simulink model "aBaja2026"  (R2026a)
settings: Solver=FixedStepAuto  StartTime=0  StopTime=1000  FixedStep=timeStep
PostLoadFcn:
  | helperSLTrajectoryFollowerWithRRScenarioSetup
InitFcn:
  | helperSLTrajectoryFollowerWithRRScenarioSetup
  | worldActor=rrSim.getScenario();
  | world = worldActor.actor_spec.world_spec;
  | % Inputs you already have (example):
  | EgoActorID  = 1;
  | egoSetSpeed = 0;
  | 
  | % Get world + actors
  | 
  | 
  | % --- Find the ego actor (vectorized, minimal overhead) ---
  | actorIDs = arrayfun(@(a) str2double(a.actor_runtime.id), world.actors);
  | idx = (actorIDs == EgoActorID);
  | 
  | if nnz(idx) ~= 1
  |     error("Actor with ActorID:%d does not exist (or is not unique).", EgoActorID);
  | end
  | 
  | ego = world.actors(idx);
  | 
  | % --- Build 4x4 pose matrix quickly ---
  | temp_m = ego.actor_runtime.pose.matrix;
  | pose = [temp_m.col0.x temp_m.col1.x temp_m.col2.x temp_m.col3.x; ...
  |         temp_m.col0.y temp_m.col1.y temp_m.col2.y temp_m.col3.y; ...
  |         temp_m.col0.z temp_m.col1.z temp_m.col2.z temp_m.col3.z; ...
  |         temp_m.col0.w temp_m.col1.w temp_m.col2.w temp_m.col3.w];
  | 
  | rotm = pose(1:3,1:3);
  | pos  = pose(1:3,4)';   % [x y z] meters
  | 
  | % --- Euler angles from rotation matrix (ZYX: yaw, pitch, roll) ---
  | % If you have Robotics System Toolbox, rotm2eul exists; otherwise keep internal.
  | if exist("rotm2eul","file")
  |     eulZYX = rotm2eul(rotm,"ZYX");                 % radians: [yaw pitch roll]
  | else
  |     eulZYX = robotics.internal.rotm2eul(rotm,"ZYX");% radians: [yaw pitch roll]
  | end
  | 
  | % RoadRunner yaw -> conventional yaw:
  | yawDeg   = rad2deg(eulZYX(1)) + 90;
  | yawDeg   = mod(yawDeg + 180, 360) - 180;           % wrap to (-180,180]
  | pitchDeg = rad2deg(eulZYX(2));
  | rollDeg  = rad2deg(eulZYX(3));
  | 
  | % --- (Optional) reproduce your actorPose struct (kept consistent) ---
  | vGlobal = [egoSetSpeed*cosd(yawDeg), egoSetSpeed*sind(yawDeg), 0];
  | vBody   = (rotm' * vGlobal')';                      % body-fixed velocity
  | 
  | actorPose = struct( ...
  |     'ActorID', double(EgoActorID), ...
  |     'Position', pos, ...
  |     'Velocity', vGlobal, ...
  |     'vehicleFrameVelocity', [vBody(2), -vBody(1), vBody(3)], ...
  |     'Roll',  rollDeg, ...
  |     'Pitch', pitchDeg, ...
  |     'Yaw',   yawDeg, ...
  |     'AngularVelocity', [0 0 0]);
  | 
  | % --- Inline replacement for poseToSim3DInputs ---
  | % IMPORTANT: your original poseToSim3DInputs uses radians (pi terms),
  | ... (+13 lines)
undefined symbols (not defined in the file): Defined, Ego, Lane, LKA, m, matlabshared, n, Pose, Sim3dSensor, timeStep, User, Velocity
libraries: roadrunnerscenario x9, drivingvehiclecontroller x3, simulink_extras x3, sim3dautolib x2, drivingscenarioandsensors x1, sim3dcameralib x1, sim3dlib x1, simulink x1
(part 2 of 2)

== system aBaja2026/LKA (Lane Keeping Assist)/Lane Source/Camera Lane Detector/Vision Lane Detector ==
  Image : Inport
  Lane Detector : MATLABSystem  System=LkaVisionLaneDetector  Vision=LKA.Vision  Ts=LKA.Ts
      mask Type: LkaVisionLaneDetector
  Processing Latency : Delay  DelayLength=LKA.Vision.LatencySteps  InitialCondition=0  SampleTime=LKA.Ts
  LaneSensor : Outport  OutDataTypeStr=Bus: LaneSensorBus
  Preview : Outport  Port=2
  VisionInfo : Outport  Port=3
  wires:
  Image/1 -> Lane Detector/1
  Lane Detector/1 -> Processing Latency/1
  Processing Latency/1 -> LaneSensor/1
  Lane Detector/2 -> Preview/1
  Lane Detector/3 -> VisionInfo/1

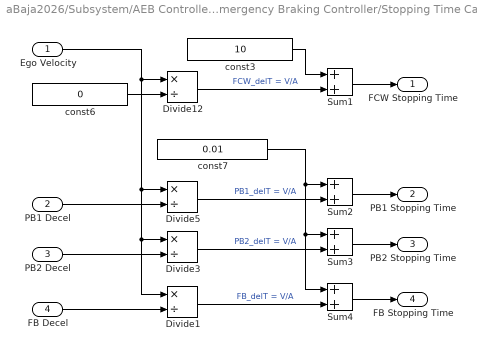
== system aBaja2026/Subsystem/AEB Controller/Emergency Braking Controller/Stopping Time Calculation ==
  Ego Velocity : Inport  SampleTime=timeStep
  PB1 Decel : Inport  Port=2
  PB2 Decel : Inport  Port=3
  FB Decel : Inport  Port=4
  Divide{1,3,5,12} (4 alike) : Product  Inputs=*/
  Sum{1..4} (4 alike) : Sum
  const3 : Constant  Value=10  SampleTime=-1
  const6 : Constant  Value=0  SampleTime=-1
  const7 : Constant  Value=0.01  SampleTime=-1
  FCW Stopping Time : Outport  VectorParamsAs1DForOutWhenUnconnected=off
  PB1 Stopping Time : Outport  Port=2  VectorParamsAs1DForOutWhenUnconnected=off
  PB2 Stopping Time : Outport  Port=3  VectorParamsAs1DForOutWhenUnconnected=off
  FB Stopping Time : Outport  Port=4  VectorParamsAs1DForOutWhenUnconnected=off
  wires:
  Sum1/1 -> FCW Stopping Time/1
  Sum2/1 -> PB1 Stopping Time/1
  Sum3/1 -> PB2 Stopping Time/1
  Sum4/1 -> FB Stopping Time/1
  const7/1 -> Sum2/1, Sum4/1, Sum3/1
  Ego Velocity/1 -> Divide1/1, Divide3/1, Divide5/1, Divide12/1
  Divide5/1 -> Sum2/2  "PB1_delT = V/A"
  Divide3/1 -> Sum3/2  "PB2_delT = V/A"
  Divide1/1 -> Sum4/2  "FB_delT = V/A"
  const6/1 -> Divide12/2
  PB1 Decel/1 -> Divide5/2
  PB2 Decel/1 -> Divide3/2
  FB Decel/1 -> Divide1/2
  const3/1 -> Sum1/1
  Divide12/1 -> Sum1/2  "FCW_delT = V/A"

== system aBaja2026/Subsystem/AEB Controller/Emergency Braking Controller/TTC Calculation ==
  Mio Distance : Inport
  Mio Velocity : Inport  Port=2
  Abs : Abs  SaturateOnIntegerOverflow=off
  Divide11 : Product  Inputs=**
  Divide3 : Product  Inputs=*/
  Saturation : Saturate  UpperLimit=100  LowerLimit=0.01
  Sign : Signum
  Sum : Sum  Inputs=+-
  const1 : Constant  Value=0  SampleTime=-1
  TTC : Outport  VectorParamsAs1DForOutWhenUnconnected=off
  wires:
  Mio Velocity/1 -> Sign/1, Abs/1
  Mio Distance/1 -> Sum/1
  Divide3/1 -> Divide11/1  "TTC"
  const1/1 -> Sum/2
  Sum/1 -> Divide3/1  "headway"
  Abs/1 -> Saturation/1
  Saturation/1 -> Divide3/2
  Sign/1 -> Divide11/2
  Divide11/1 -> TTC/1

== matlab function aBaja2026/Subsystem2/MATLAB Function1 ==
  data: T input; Translation output; Rotation output
function [Translation, Rotation] = poseToSim3DInputs(T)
% T: 4x4 pose matrix
% Outputs:
%   Translation - 5x3 matrix
%   Rotation    - 5x3 matrix

% ------------------------------------------
% 1. Extract vehicle translation
% ------------------------------------------
Xv = T(1,4);
Yv = -1*T(2,4);
Zv = T(3,4);

% ------------------------------------------
% 2. Extract vehicle yaw (ISO 8855, Z-down)
% ------------------------------------------
yaw = atan2(T(2,1), T(1,1));    % heading
roll = 0;                       % assume level (modify if needed)
pitch = 0;

% ------------------------------------------
% 3. Build Translation 5×3
% Row 1 = vehicle
% Rows 2–5 = wheels (zero unless user fills)
% ------------------------------------------
Translation = zeros(5,3);
Translation(1,:) = [Xv, Yv, Zv];

% ------------------------------------------
% 4. Build Rotation 5×3
% Row 1 = vehicle rotation
% Rows 2–5 = wheels
% ------------------------------------------
Rotation = zeros(5,3);
Rotation(1,:) = [roll, pitch, -yaw+pi/2+pi];

== matlab function aBaja2026/Subsystem2/Pack Actor Pose/Velocity XYZ Components ==
  data: yaw input size=1; velocity output size=[1 3]; speed input size=1
function velocity = computeVelocity(yaw, speed)

% Output velocity vector (x,y,z)
velocity = speed * [-sind(yaw) cosd(yaw) 0];

== matlab function aBaja2026/Subsystem2/Lateral Metrics ==
  data: currPose input size=[1 3]; refPose input size=[1 3]; positionError output; headingError output
function [positionError, headingError] = lateralMetrics(currPose, refPose)
%lateralMetrics calculates lateral error and heading error of the vehicle 
% using current and reference pose

currPose(:,3) = deg2rad(currPose(:,3));
refPose(:,3)  = deg2rad(refPose(:,3));

positionError = norm(currPose(1:2) - refPose(1:2));

headingError = rad2deg(currPose(:, 3) - refPose(:,3));

== matlab function aBaja2026/LKA (Lane Keeping Assist)/Skeleton Pose Adapter ==
  data: veh input Bus: BusVehicleInfo; egoPose output; refPose input; refCurv input; mode input; centerPose output; curv output; speed output; yawRate output; enable output; yawRatePose output; LKA parameter
function [egoPose, centerPose, curv, speed, yawRate, enable, yawRatePose] = fcn(veh, refPose, refCurv, mode, LKA)
% Skeleton signals -> LKA conventions (SI units, radians, rear-axle reference).
% speed / yawRate stand for the wheel-speed sensor and the gyro (noise added by the
% Ego Sensors block). egoPose, centerPose, curv feed only the emulated sensor
% (development variant). yawRatePose is differentiated from the ground-truth pose
% and only logged to verify LKA.Cosim.YawRateSign (rule I.2.3: not a controller input).
persistent psiPrev
psi = deg2rad(veh.CurrPose(3) + LKA.Cosim.YawOffsetDeg);
if isempty(psiPrev), psiPrev = psi; end
yawRatePose = lka_wrap_angle(psi - psiPrev) / LKA.Ts;
psiPrev = psi;
yawRate = LKA.Cosim.YawRateSign * deg2rad(veh.CurrYawRate);
egoPose = [veh.CurrPose(1) + LKA.Cosim.PoseToRearAxle*cos(psi), ...
           veh.CurrPose(2) + LKA.Cosim.PoseToRearAxle*sin(psi), psi];
centerPose = [refPose(1), refPose(2), deg2rad(refPose(3) + LKA.Cosim.YawOffsetDeg)];
curv = [refCurv(1), 0];
speed = abs(veh.CurrVelocity);
enable = any(mode == LKA.Cosim.LkaModes);

== matlab function aBaja2026/Subsystem2/Initialize State/Calculate Initial States/Calculate Initial States ==
  data: egoRuntime input; egoInitialState output Bus: BusVehicleInfo
function egoInitialState = getInitialState(egoRuntime)
%getInitialState calculates initial conditions of the vehicle

% Calculate velocity
velocity = norm(egoRuntime.ActorRuntime.Velocity,2);
% Get Transformation matrix
transformationMatrix = egoRuntime.ActorRuntime.Pose;
% Get pose information
x = transformationMatrix(1,4);
y = transformationMatrix(2,4);
yaw = atan2d(-transformationMatrix(1,2), ...
            transformationMatrix(1,1));
% Pack the initial states
egoInitialState = struct('CurrPose', [y, -x, yaw], ...
    'CurrVelocity', velocity, ...
    'CurrYawRate', 0, ...
    'CurrSteer',0, ...
    'Direction',1);

== matlab function aBaja2026/Subsystem/AEB Controller/Ego Speed ==
  data: speed output; velocity input
function speed = egoSpeed(velocity)

speed = norm([velocity(1), velocity(2), velocity(3)]);

== stateflow chart aBaja2026/Subsystem/AEB Controller/Emergency Braking Controller/AEB Logic ==
  note: FCW/AEB Logic
  state Default
    entry: AEBstatus = 0;
    FCWactivate = 0;
    decel = 0;
  state FCW
    entry: AEBstatus = 0;
    FCWactivate = 1;
    decel = 0;
  state Partial_Braking1
    entry: AEBstatus = 1;
    FCWactivate = 1;
    decel = PB1decel;
  state Full_Braking
    entry: AEBstatus = 3;
    FCWactivate = 1;
    decel = FBdecel;
  state Partial_Braking2
    entry: AEBstatus = 2;
    FCWactivate = 1;
    decel = PB2decel;
  (default) -> Default
  (junction 78) -> Default
  Full_Braking -> (junction 78) [order 1] : [stop==1]
  (junction 80) -> Default
  (junction 90) -> (junction 80) : [stop==1]
  (junction 86) -> Default
  (junction 88) -> (junction 86)
  Default -> FCW : [(abs(TTC)<FCWtime) && TTC<0&&stop~=1]
  FCW -> (junction 76) [order 1]
  (junction 76) -> Full_Braking : [ abs(relativeYawAngle) >= deg2rad(89) && TTC<0 && ...
      | stop~=1]
  FCW -> Partial_Braking1 [order 2] : [(abs(TTC) < PB1time) && TTC<0&&stop~=1]
  Partial_Braking1 -> (junction 88) [order 2] : [stop==1]
  Partial_Braking1 -> Partial_Braking2 [order 1] : [(abs(TTC) < PB2time) && TTC<0&&stop~=1]
  Partial_Braking2 -> Partial_Braking1 [order 2] : [abs(TTC)>=1.2*PB2time]
  Partial_Braking2 -> (junction 90) [order 1]
  Full_Braking -> Partial_Braking2 [order 2] : [abs(TTC)>=3*FBtime]
  Partial_Braking2 -> Full_Braking [order 3] : [(abs(TTC) < FBtime) && TTC<0&&stop~=1]
  data: FCWactivate output uint8; TTC input; FCWtime input; PB1time input; PB2time input; FBtime input; PB1decel input; PB2decel input; FBdecel input; AEBstatus output uint8; decel output; stop input; relativeYawAngle input

== matlab function aBaja2026/Subsystem/AEB Controller/Find MIO ==
  data: confirmedTracks input size=[1 1]; x output size=[1 1]; vx output size=[1 1]; positionSelector input; laneWidth input; relativeYawAngle output double size=[1 1]; egoSpeed input double size=[1 1]
function [x,vx, relativeYawAngle] = findMIO(confirmedTracks, positionSelector, laneWidth, egoSpeed)
% This function finds the lead car: a car in front of the ego car that
% satisfies all the criteria below:
% * Within the ego car's lane.
% * In front of the ego car.
% * Closest to the ego car.

% Important notes:
% 1. If you change state definition, change the following:
%       State = [x;vx;y;vy;z;vz] (3D constant velocity)
numStates = 6;
relativeYawAngle =0 ;
% 2. The ego car is assumed to be traveling in the middle of its lane.
halfLaneWidth = laneWidth/2;

% Initialize outputs and parameters
maxX = cast(1000, 'like', confirmedTracks.Tracks(1).State);  % Far enough forward so that no track is expected to exceed this distance
trackID = 0;
crossingTargetLateralDist = 18;
targetCollisionThresholdTime = 2; % Collision threshold time beyond which the target should be treated as MIO 
stationaryVelocityThreshold = eps('single'); % Threshold to determine if a target is effectively stationary relative to the world

for i = 1:confirmedTracks.NumTracks
    position = positionSelector * confirmedTracks.Tracks(i).State;
    x = position(1); % Longitudinal position of the track relative to ego
    y = position(2); % Lateral position of the track relative to ego

    if x < maxX && x > 0 % No point checking otherwise
        % Detect cross target as MIO to avoid collision
        
        if (-crossingTargetLateralDist <= y) && (y <= crossingTargetLateralDist) &&  ...
                abs(norm([confirmedTracks.Tracks(i).State(2), confirmedTracks.Tracks(i).State(4), confirmedTracks.Tracks(i).State(6)]) - egoSpeed) >= stationaryVelocityThreshold
            estimatedCollisionTime = confirmedTracks.Tracks(i).State(1)/abs(confirmedTracks.Tracks(i).State(2));
            if(targetCollisionThresholdTime>abs(estimatedCollisionTime))
                maxX = x;
                trackID = i;
            end
        end

        yleftLane  = polyval([0, 0,  halfLaneWidth],x); % Half a lane to the left
        yrightLane = polyval([0, 0, -halfLaneWidth],x); % Half a lane to the right
        % Find a new lead car
        if (yrightLane <= y) && (y <= yleftLane)
            maxX = x;
            trackID = i;
        end
    end
end

if trackID>0
    mioState = confirmedTracks.Tracks(trackID).State;
    relativeYawEgoFrame = atan2(mioState(4), mioState(2));
    relativeYawAngle = relativeYawEgoFrame;
else
    mioState = zeros(numStates,1,'like',confirmedTracks.Tracks(1).State);
    mioState(1) = 500;
    mioState(2) = 0.01;
end

% Output:
x = mioState(1);    % Longitudinal position of the lead car
vx = mioState(2);   % Longitudinal velocity of the lead car

== matlab function aBaja2026/Subsystem/MATLAB Function ==
  data: u input; y output
function y = fcn(u)

y = norm(u);

== matlab function aBaja2026/LKA (Lane Keeping Assist)/Ego Sensors (wheel speed + IMU)/Sensor Model ==
  data: v input; vMeas output; r input; n input; rMeas output; LKA parameter
function [vMeas, rMeas] = fcn(v, r, n, LKA)
% Wheel-speed sensor and gyro with scale error, bias and noise (lka_ego_sensor_model.m)
[vMeas, rMeas] = lka_ego_sensor_model(v, r, n, LKA.EgoSen);

== matlab function aBaja2026/Subsystem2/Pack Actor Pose/Pose Generation ==
  data: pose input; currPose output
function currPose = generatePose(pose)

yaw = deg2rad(pose(3));
rotm = eul2rotm([yaw 0 0]);

currPose = [[rotm [pose(1:2) 0]']; [0 0 0 1]];
